simulink model "simulink_file"  (R2022b)
settings: Solver=ode45  StartTime=0.0  StopTime=2  RelTol=1e-3  EnableMultiTasking=on
libraries: spsCurrentMeasurementLib x7, spsMosfetLib x7, spsSeriesRLCBranchLib x6, spsDCVoltageSourceLib x1, spsVoltageMeasurementLib x1, sps_lib x1
settings Model: Creator=dhanu  LastModifiedBy=dell
settings SolverCC: AlgebraicLoopSolver=TrustRegion
settings DataIOCC: LimitDataPoints=on  SaveFormat=Array  SignalLoggingSaveFormat=ModelDataLogs  ReturnWorkspaceOutputs=off
settings OptimizationCC: ExpressionDepthLimit=2147483647  LifeSpan=inf
settings DebuggingCC: UnderspecifiedInitializationDetection=Classic  MergeDetectMultiDrivingBlocksExec=none  SolverPrmCheckMsg=warning  FcnCallInpInsideContextMsg=warning  UnconnectedInputMsg=warning  UnconnectedOutputMsg=warning  UnconnectedLineMsg=warning  StateNameClashWarn=warning  SFUnexpectedBacktrackingDiag=warning  SFNoUnconditionalDefaultTransitionDiag=warning  SFExecutionAtInitializationDiag=none  SFMachineParentedDataDiag=warning  ArithmeticOperatorsInVariantConditions=warning
settings HardwareCC: ProdBitPerPointer=32  ProdBitPerSizeT=32  ProdBitPerPtrDiffT=32  ProdLargestAtomicFloat=None  ProdIntDivRoundTo=Undefined  ProdEndianess=Unspecified  ProdWordSize=32  ProdHWDeviceType=32-bit Generic
settings ModelReferenceCC: PropagateSignalLabelsOutOfModel=off
settings SFSimCC: SimUseLocalCustomCode=off  CustomCodeUndefinedFunction=UseInterfaceOnly
settings RTWCC: RTWUseLocalCustomCode=off
settings CodeAppCC: StateflowObjectComments=on
settings GRTTargetCC: TargetLangStandard=C89/C90 (ANSI)  CombineOutputUpdateFcns=off  GRTInterface=on
settings ConfigComp: CovMetricSettings=dw  CovSaveCumulativeToWorkspaceVar=on  CovSaveSingleToWorkspaceVar=on  CovExternalEMLEnable=off
settings SimscapeCC: SimscapeNormalizeSystem=off

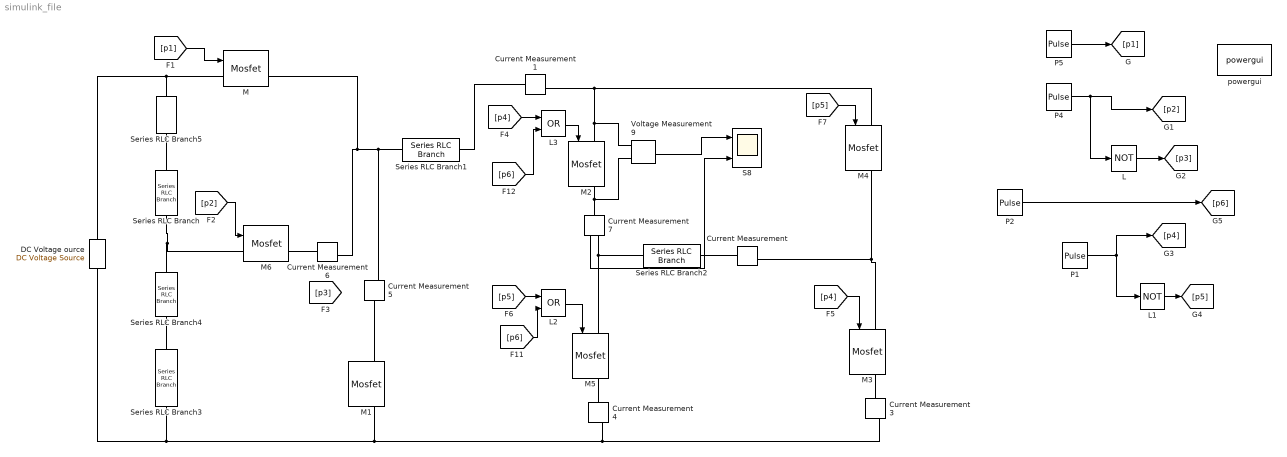
== system simulink_file ==
  Current Measurement{,1,3..7} (7 alike) : spsCurrentMeasurementLib/Current Measurement  PhasorSimulation=off  OutputType=Complex  PSBequivalent=0
  DC Voltage ource : spsDCVoltageSourceLib/DC Voltage Source  Amplitude=75  Measurements=None
  L : Logic  Operator=NOT  AllPortsSameDT=off  OutDataTypeStr=boolean
  L1 : Logic  Operator=NOT  AllPortsSameDT=off  OutDataTypeStr=boolean
  L2 : Logic  Operator=OR  AllPortsSameDT=off  OutDataTypeStr=boolean
  L3 : Logic  Operator=OR  AllPortsSameDT=off  OutDataTypeStr=boolean
  M{,1..6} (7 alike) : spsMosfetLib/Mosfet  Ron=0.1  Lon=0  Rd=0.01  Vfd=0  IC=0  Rs=1e5  Cs=inf  Measurements=on
  P1 : DiscretePulseGenerator  PulseType=Time based  Period=1/50  PulseWidth=50
  P2 : DiscretePulseGenerator  PulseType=Time based  Period=0.01  PulseWidth=2.5  PhaseDelay=0.00005
  P4 : DiscretePulseGenerator  PulseType=Time based  Period=0.01  PulseWidth=69  PhaseDelay=0.00056
  P5 : DiscretePulseGenerator  PulseType=Time based  Period=0.01  PulseWidth=33  PhaseDelay=0.0018
  S8 : Scope  NumInputPorts=2
  Series RLC Branch : spsSeriesRLCBranchLib/Series RLC Branch  LConnTagsString=__new0  RConnTagsString=__new0  BranchType=C  Resistance=1  Inductance=1e-3  SetiL0=off  InitialCurrent=0  Capacitance=600e-6  Setx0=off  InitialVoltage=0  Measurements=None
  Series RLC Branch1 : spsSeriesRLCBranchLib/Series RLC Branch  LConnTagsString=__new0  RConnTagsString=__new0  BranchType=L  Resistance=1  Inductance=14e-3  SetiL0=off  InitialCurrent=0  Capacitance=1e-6  Setx0=off  InitialVoltage=0  Measurements=None
  Series RLC Branch2 : spsSeriesRLCBranchLib/Series RLC Branch  LConnTagsString=__new0  RConnTagsString=__new0  BranchType=R  Resistance=12  Inductance=0.01e-3  SetiL0=off  InitialCurrent=0  Capacitance=1e-6  Setx0=off  InitialVoltage=0  Measurements=None
  Series RLC Branch3 : spsSeriesRLCBranchLib/Series RLC Branch  LConnTagsString=__new0  RConnTagsString=__new0  BranchType=C  Resistance=1  Inductance=1e-3  SetiL0=off  InitialCurrent=0  Capacitance=600e-6  Setx0=off  InitialVoltage=0  Measurements=None
  Series RLC Branch4 : spsSeriesRLCBranchLib/Series RLC Branch  LConnTagsString=__new0  RConnTagsString=__new0  BranchType=R  Resistance=2.8  Inductance=1e-3  SetiL0=off  InitialCurrent=0  Capacitance=1000e-6  Setx0=off  InitialVoltage=0  Measurements=None
  Series RLC Branch5 : spsSeriesRLCBranchLib/Series RLC Branch  LConnTagsString=__new0  RConnTagsString=__new0  BranchType=R  Resistance=2.8  Inductance=1e-3  SetiL0=off  InitialCurrent=0  Capacitance=1000e-6  Setx0=off  InitialVoltage=0  Measurements=None
  Voltage Measurement9 : spsVoltageMeasurementLib/Voltage Measurement  PhasorSimulation=off  OutputType=Complex  PSBequivalent=0
  powergui : sps_lib/powergui  Priority=1  SimulationMode=Discrete  SampleTime=5e-5  frequency=60  Iterations=50  frequencyindice=0  Pbase=100e6  ErrMax=1e-4  UnitsV=kV  UnitsW=MW  buscounter=0  FunctionMessages=off  echomessages=off  EnableUseOfTLC=off  CurrentSourceSwitches=off  DisableSnubberDevices=off  DisableRonSwitches=off  DisableVfSwitches=off  DisplayEquations=off  AutomaticDiscreteSolvers=off  SolverType=Tustin  Interpol=off  ExternalGateDelay=off  methode=off  Ts=0  x0status=blocks  SPID=off  SwTol=0  HookPort=off  NonlinearTolerance=1e-4  nMaxIteration=100  ContinueOnMaxIteration=off  RestoreLinks=warning  ResistiveCurrentMeasurement=off  Frange=[0:2:500]  Ylog=off  Xlog=on  ShowGrid=off  save=off  variable=ZData  structure=vol  ZoomFFT=off  StartTime=1.98  cycles=1  DisplayStyle=1  fundamental=50  FreqAxis=off  MaxFrequency=1000  frequencyindicesteady=1  RmsSteady=1  display=off
  wires:
  P5/1 -> [p1]
  P4/1 -> L/1, [p2]
  L/1 -> [p3]
  P1/1 -> [p4], L1/1
  L1/1 -> [p5]
  [p1] -> M/1
  [p2] -> M6/1
  [p5] -> M4/1
  [p4] -> M3/1
  [p4] -> L3/1
  [p6] -> L3/2
  L3/1 -> M2/1
  L2/1 -> M5/1
  [p5] -> L2/1
  [p6] -> L2/2
  P2/1 -> [p6]
  Voltage Measurement9/1 -> S8/1
  Current Measurement7/1 -> S8/2
  connections:
  M2/LConn1 -- Voltage Measurement9/LConn1 -- M4/LConn1 -- Current Measurement1/RConn1
  DC Voltage ource/LConn1 -- Series RLC Branch3/RConn1 -- M1/RConn1 -- Current Measurement4/RConn1 -- Current Measurement3/RConn1
  Current Measurement/LConn1 -- Series RLC Branch2/RConn1
  M/LConn1 -- DC Voltage ource/RConn1 -- Series RLC Branch5/LConn1
  M6/LConn1 -- Series RLC Branch/RConn1 -- Series RLC Branch4/LConn1
  Series RLC Branch4/RConn1 -- Series RLC Branch3/LConn1
  Series RLC Branch5/RConn1 -- Series RLC Branch/LConn1
  Current Measurement1/LConn1 -- Series RLC Branch1/RConn1
  Series RLC Branch2/LConn1 -- M5/LConn1 -- Current Measurement7/RConn1
  M3/LConn1 -- M4/RConn1 -- Current Measurement/RConn1
  Current Measurement7/LConn1 -- Voltage Measurement9/LConn2 -- M2/RConn1
  Current Measurement3/LConn1 -- M3/RConn1
  Current Measurement4/LConn1 -- M5/RConn1
  Current Measurement5/LConn1 -- M1/LConn1
  Current Measurement6/LConn1 -- M6/RConn1
  Series RLC Branch1/LConn1 -- M/RConn1 -- Current Measurement6/RConn1 -- Current Measurement5/RConn1
